simulink library "tailsitter_lib"  (R2018b)
settings: Solver=VariableStepAuto  StartTime=0.0  StopTime=10.0  RelTol=1e-3
undefined symbols (not defined in the file or in its folder): envir, tailsitter
libraries: unit_conversions_lib x2, simple_wing_lib x2, propulsion_lib x2, rotorcraft_lib x2, actuators_lib x2, flightgear_visualization_lib x1, simpleFuselage_lib x1, ground_lib x1, rigidBody_lib x1
settings Model: Creator=Ybeyer  LastModifiedBy=yannic
settings SFSimCC: SimUseLocalCustomCode=off
settings RTWCC: RTWUseLocalCustomCode=off
settings CodeAppCC: StateflowObjectComments=on

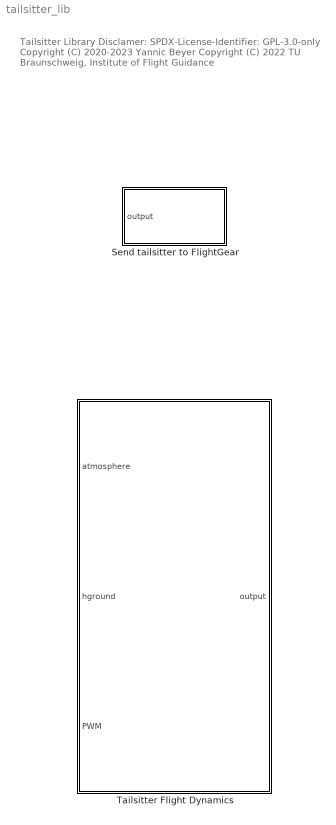
== system tailsitter_lib ==
  note: Tailsitter Library
      |
      | Disclamer:
      | SPDX-License-Identifier: GPL-3.0-only
      |
      | Copyright (C) 2020-2023 Yannic Beyer
      | Copyright (C) 2022 TU Braunschweig, Institute of Flight Guidance
  Send tailsitter to FlightGear : Subsystem  mask{posRef=tailsitter.posRef, IP='127.0.0.1', Port=5502}
      mask prompts: posRef "reference position struct"; IP "FlightGear receive IP"; Port "FlightGear receive Port"
      mask DialogControl DescGroupVar Prompt: Send tailsitter to FlightGear
      mask DialogControl DescTextVar Prompt: Connect the output of the Tailsitter Flight Dynamics block to this block and run a tailsitter FlightGear start script.
  Tailsitter Flight Dynamics : Subsystem  mask{tailsitter=tailsitter}
      mask prompts: tailsitter "tailsitter parameters struct"
      mask DialogControl DescGroupVar Prompt: Tailsitter Flight Dynamics
      mask DialogControl DescTextVar Prompt: For more information about the tailsitter parameters struct see tailsitterLoadParams.

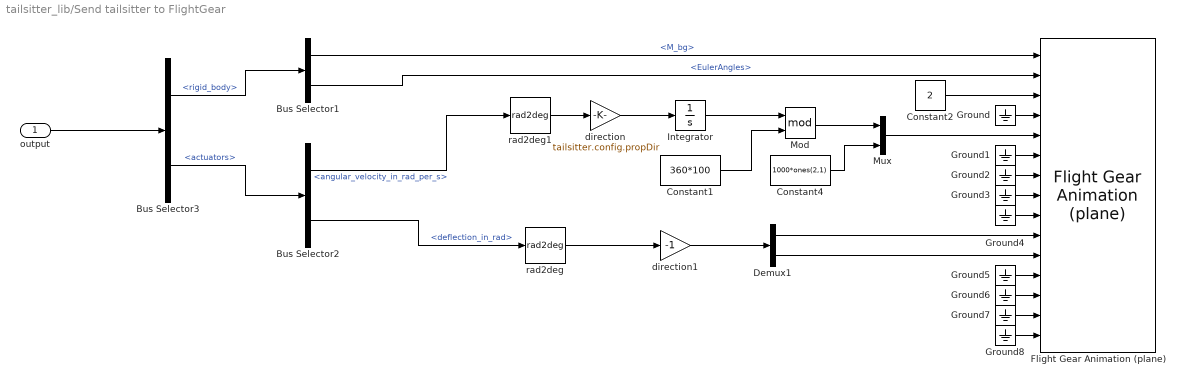
== system tailsitter_lib/Send tailsitter to FlightGear ==
  output : Inport
  Bus Selector1 : BusSelector  OutputSignals=M_bg,EulerAngles
  Bus Selector2 : BusSelector  OutputSignals=angular_velocity_in_rad_per_s,eta_i.deflection_in_rad
  Bus Selector3 : BusSelector  OutputSignals=rigid_body,actuators
  Constant1 : Constant  Value=360*100
  Constant2 : Constant  Value=2
  Constant4 : Constant  Value=1000*ones(2,1)
  Demux1 : Demux  Outputs=2
  Flight Gear Animation (plane) : flightgear_visualization_lib/Flight Gear Animation (plane)  inital_lat=posRef.lat  inital_long=posRef.lon  inital_height=posRef.alt  remoteURL=IP  remotePort=Port
      settings: SourceProductName=LADAC
  Ground{,1..8} (9 alike) : Ground
  Integrator : Integrator
  Mod : Math  Operator=mod  SaturateOnIntegerOverflow=on
  Mux : Mux  Inputs=2
  direction : Gain  Gain=tailsitter.config.propDir
  direction1 : Gain  Gain=-1
  rad2deg : unit_conversions_lib/rad2deg
      settings: SourceProductName=LADAC
  rad2deg1 : unit_conversions_lib/rad2deg
      settings: SourceProductName=LADAC
  wires:
  direction1/1 -> Demux1/1
  Constant4/1 -> Mux/2
  Ground/1 -> Flight Gear Animation (plane)/4
  Demux1/2 -> Flight Gear Animation (plane)/11
  Bus Selector1/2 -> Flight Gear Animation (plane)/2  "<EulerAngles>"
  Demux1/1 -> Flight Gear Animation (plane)/10
  rad2deg1/1 -> direction/1
  Bus Selector1/1 -> Flight Gear Animation (plane)/1  "<M_bg>"
  Ground1/1 -> Flight Gear Animation (plane)/6
  Bus Selector2/2 -> rad2deg/1  "<deflection_in_rad>"
  Bus Selector2/1 -> rad2deg1/1  "<angular_velocity_in_rad_per_s>"
  direction/1 -> Integrator/1
  Mod/1 -> Mux/1
  Integrator/1 -> Mod/1
  Constant1/1 -> Mod/2
  Mux/1 -> Flight Gear Animation (plane)/5
  Constant2/1 -> Flight Gear Animation (plane)/3
  Ground4/1 -> Flight Gear Animation (plane)/9
  rad2deg/1 -> direction1/1
  output/1 -> Bus Selector3/1
  Ground7/1 -> Flight Gear Animation (plane)/14
  Ground6/1 -> Flight Gear Animation (plane)/13
  Ground8/1 -> Flight Gear Animation (plane)/15
  Ground5/1 -> Flight Gear Animation (plane)/12
  Ground2/1 -> Flight Gear Animation (plane)/7
  Ground3/1 -> Flight Gear Animation (plane)/8
  Bus Selector3/1 -> Bus Selector1/1  "<rigid_body>"
  Bus Selector3/2 -> Bus Selector2/1  "<actuators>"

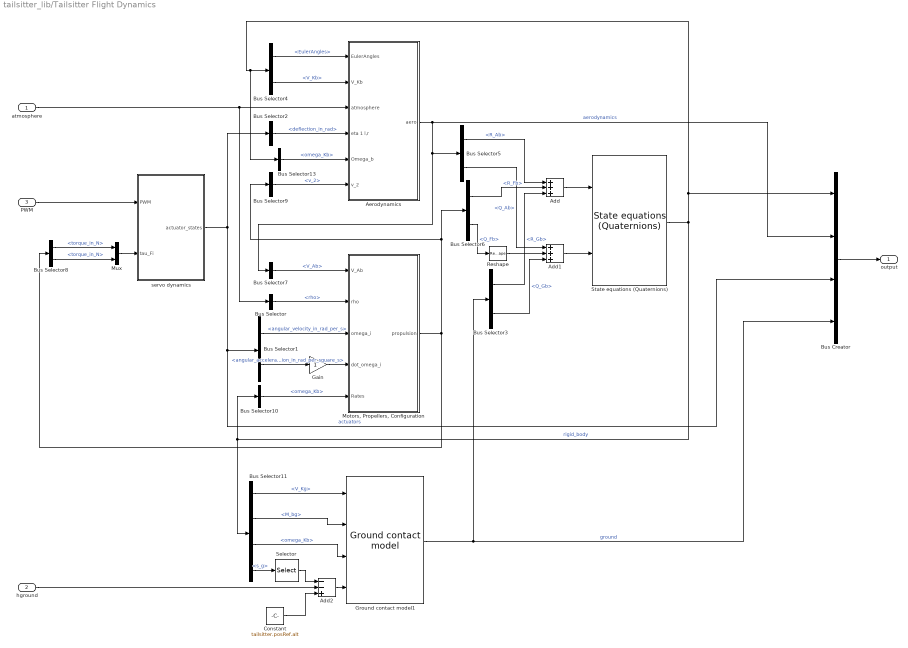
== system tailsitter_lib/Tailsitter Flight Dynamics ==
  atmosphere : Inport
  hground : Inport  Port=2
  PWM : Inport  Port=3
  Add : Sum  Inputs=3
  Add1 : Sum  Inputs=3
  Add2 : Sum  Inputs=--+
  Aerodynamics : Subsystem
  Bus Creator : BusCreator  Inputs=4
  Bus Selector : BusSelector  OutputSignals=athmosphere.rho
  Bus Selector1 : BusSelector  OutputSignals=angular_velocity_in_rad_per_s,angular_acceleration_in_rad_per_square_s
  Bus Selector10 : BusSelector  OutputSignals=omega_Kb
  Bus Selector11 : BusSelector  OutputSignals=V_Kg,M_bg,omega_Kb,s_g
  Bus Selector13 : BusSelector  OutputSignals=omega_Kb
  Bus Selector2 : BusSelector  OutputSignals=eta_i.deflection_in_rad
  Bus Selector3 : BusSelector  OutputSignals=forces_and_moments.R_Gb,forces_and_moments.Q_Gb
  Bus Selector4 : BusSelector  OutputSignals=EulerAngles,V_Kb
  Bus Selector5 : BusSelector  OutputSignals=cg aerodynamics.R_Ab,cg aerodynamics.Q_Ab
  Bus Selector6 : BusSelector  OutputSignals=R_Fb,Q_Fb
  Bus Selector7 : BusSelector  OutputSignals=cg aerodynamics.aeroAxes.V_Ab
  Bus Selector8 : BusSelector  OutputSignals=prop_1.torque_in_N,prop_2.torque_in_N
  Bus Selector9 : BusSelector  OutputSignals=v_2
  Constant : Constant  Value=tailsitter.posRef.alt
  Gain : Gain
  Ground contact model1 : ground_lib/Ground contact model  m=tailsitter.body.m  a_max=tailsitter.grnd.acc_max  xyz_c_hit=tailsitter.config.hitPoints_c  xyz_c_cg=tailsitter.config.CoG_Pos_c  ground_softness_param=tailsitter.grnd.softness_parameter  k_h=tailsitter.grnd.spring_stiffness  k_dot_h=tailsitter.grnd.damping  mu=tailsitter.grnd.friction_coef  k_V=tailsitter.grnd.low_speed_friction_reduction_factor
      settings: SourceProductName=LADAC
  "Motors, Propellers, Configuration" : Subsystem
  Mux : Mux  Inputs=2
  Reshape : Reshape  OutputDimensionality=Column vector (2-D)
  Selector : Selector  InputPortWidth=3  IndexOptions=Index vector (dialog)  Indices=3  OutputSizes=1
  State equations (Quaternions) : rigidBody_lib/State equations (Quaternions)  m=tailsitter.body.m  I=tailsitter.body.I  is_g_checked=off  g=envir.g  omega_Kb_0=tailsitter.ic.omega_kb_b  q_bg_0=tailsitter.ic.q_bg  V_Kb_0=tailsitter.ic.V_kb_b  s_g_0=tailsitter.ic.s_g
      settings: SourceProductName=LADAC
  servo dynamics : Subsystem
  output : Outport
  wires:
  PWM/1 -> servo dynamics/1(PWM)
  atmosphere/1 -> Bus Selector/1, Aerodynamics/3(atmosphere)
  Bus Selector/1 -> "Motors, Propellers, Configuration"/2(rho)  "<rho>"
  servo dynamics/1(actuator_states) -> Bus Creator/3, Bus Selector1/1, Bus Selector2/1  "actuators"
  Bus Selector1/1 -> "Motors, Propellers, Configuration"/3("omega_i ")  "<angular_velocity_in_rad_per_s>"
  Bus Selector1/2 -> Gain/1  "<angular_acceleration_in_rad_per_square_s>"
  Bus Selector2/1 -> Aerodynamics/4(eta 1 l,r)  "<deflection_in_rad>"
  Bus Selector5/1 -> Add/1  "<R_Ab>"
  Bus Selector5/2 -> Add1/1  "<Q_Ab>"
  Bus Selector6/2 -> Reshape/1  "<Q_Fb>"
  Bus Selector6/1 -> Add/2  "<R_Fb>"
  "Motors, Propellers, Configuration"/1(propulsion) -> Bus Selector8/1, Bus Selector9/1, Bus Selector6/1
  Bus Selector7/1 -> "Motors, Propellers, Configuration"/1(V_Ab)  "<V_Ab>"
  Bus Selector8/1 -> Mux/1  "<torque_in_N>"
  Bus Selector9/1 -> Aerodynamics/6(v_2)  "<v_2>"
  Gain/1 -> "Motors, Propellers, Configuration"/4(dot_omega_i)
  Ground contact model1/1 -> Bus Selector3/1, Bus Creator/4  "ground"
  Add1/1 -> State equations (Quaternions)/2
  hground/1 -> Add2/2
  Bus Creator/1 -> output/1
  Add/1 -> State equations (Quaternions)/1
  Aerodynamics/1(aero) -> Bus Selector7/1, Bus Selector5/1, Bus Creator/2  "aerodynamics"
  State equations (Quaternions)/1 -> Bus Selector13/1, Bus Selector4/1, Bus Creator/1, Bus Selector11/1, Bus Selector10/1  "rigid_body"
  Bus Selector4/1 -> Aerodynamics/1("EulerAngles ")  "<EulerAngles>"
  Bus Selector4/2 -> Aerodynamics/2(V_Kb)  "<V_Kb>"
  Bus Selector10/1 -> "Motors, Propellers, Configuration"/5("Rates ")  "<omega_Kb>"
  Bus Selector11/4 -> Selector/1  "<s_g>"
  Bus Selector11/3 -> Ground contact model1/3  "<omega_Kb>"
  Bus Selector11/2 -> Ground contact model1/2  "<M_bg>"
  Bus Selector11/1 -> Ground contact model1/1  "<V_Kg>"
  Bus Selector13/1 -> Aerodynamics/5(Omega_b)  "<omega_Kb>"
  Bus Selector3/2 -> Add1/3  "<Q_Gb>"
  Bus Selector3/1 -> Add/3  "<R_Gb>"
  Reshape/1 -> Add1/2
  Add2/1 -> Ground contact model1/4
  Selector/1 -> Add2/1
  Constant/1 -> Add2/3
  Mux/1 -> servo dynamics/2(tau_Fi)
  Bus Selector8/2 -> Mux/2  "<torque_in_N>"

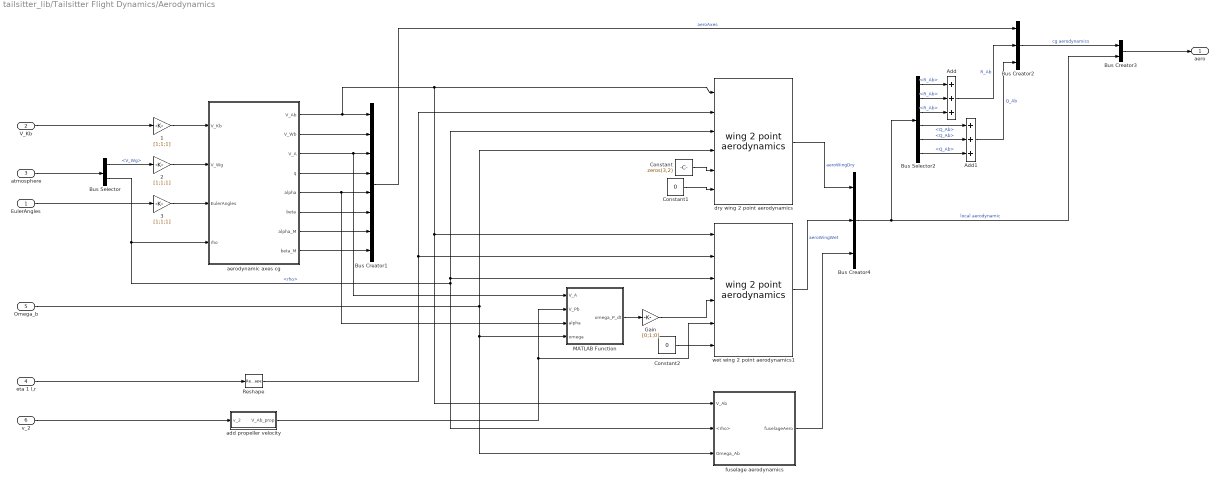
== system tailsitter_lib/Tailsitter Flight Dynamics/Aerodynamics ==
  "EulerAngles " : Inport
  V_Kb : Inport  Port=2
  atmosphere : Inport  Port=3
  eta 1 l,r : Inport  Port=4
  Omega_b : Inport  Port=5
  v_2 : Inport  Port=6
  1 : Gain  Gain=[1;1;1]
  2 : Gain  Gain=[1;1;1]  OutDataTypeStr=double
  3 : Gain  Gain=[1;1;1]
  Add : Sum  Inputs=+++
  Add1 : Sum  Inputs=+++
  Bus Creator1 : BusCreator  Inputs=8
  Bus Creator2 : BusCreator  Inputs=3
  Bus Creator3 : BusCreator  Inputs=2
  Bus Creator4 : BusCreator  Inputs=3
  Bus Selector : BusSelector  OutputSignals=V_Wg,athmosphere.rho
  Bus Selector2 : BusSelector  OutputSignals=aeroWingDry.dynamicsBody.R_Ab,aeroWingWet.dynamicsBody.R_Ab,aeroFuselage.dynamics.R_Ab,aeroWingDry.dynamicsBody.Q_Ab,aeroWingWet.dynamicsBody.Q_Ab,aeroFuselage.dynamics.Q_Ab
  Constant : Constant  Value=zeros(3,2)
  Constant1 : Constant  Value=0
  Constant2 : Constant  Value=0
  Gain : Gain  Gain=[0;1;0]
  MATLAB Function : MATLAB Function  TreatAsAtomicUnit=on
  Reshape : Reshape  OutputDimensionality=Row vector (2-D)
  add propeller velocity : MATLAB Function  TreatAsAtomicUnit=on
  aerodynamic axes cg : MATLAB Function  TreatAsAtomicUnit=on
  dry wing 2 point aerodynamics : simple_wing_lib/wing 2 point aerodynamics  wingStruct=tailsitter.aero.wing  xyz_wing_c=tailsitter.config.xyz_c_wing  xyz_cg_c=tailsitter.config.CoG_Pos_c
      settings: SourceProductName=LADAC
  fuselage aerodynamics : Subsystem  mask{simple_fuselage=tailsitter.aero.fuse}
      mask prompts: simple_fuselage "fuselage struct"
  wet wing 2 point aerodynamics1 : simple_wing_lib/wing 2 point aerodynamics  wingStruct=tailsitter.aero.wing_wet  xyz_wing_c=tailsitter.config.xyz_c_wing  xyz_cg_c=tailsitter.config.CoG_Pos_c
      settings: SourceProductName=LADAC
  aero : Outport
  wires:
  atmosphere/1 -> Bus Selector/1
  Bus Selector/1 -> 2/1  "<V_Wg>"
  2/1 -> aerodynamic axes cg/2(V_Wg)
  "EulerAngles "/1 -> 3/1
  1/1 -> aerodynamic axes cg/1(V_Kb)
  V_Kb/1 -> 1/1
  3/1 -> aerodynamic axes cg/3(EulerAngles)
  aerodynamic axes cg/1(V_Ab) -> Bus Creator1/1, dry wing 2 point aerodynamics/1, fuselage aerodynamics/1(V_Ab), wet wing 2 point aerodynamics1/1
  Bus Selector/2 -> fuselage aerodynamics/2(<rho>), dry wing 2 point aerodynamics/3, wet wing 2 point aerodynamics1/3, aerodynamic axes cg/4(rho)  "<rho>"
  eta 1 l,r/1 -> Reshape/1
  v_2/1 -> add propeller velocity/1(v_2)
  aerodynamic axes cg/2(V_Wb) -> Bus Creator1/2
  aerodynamic axes cg/3(V_A) -> MATLAB Function/1(V_A), Bus Creator1/3
  aerodynamic axes cg/4(q) -> Bus Creator1/4
  aerodynamic axes cg/5(alpha) -> MATLAB Function/3(alpha), Bus Creator1/5
  aerodynamic axes cg/6(beta) -> Bus Creator1/6
  aerodynamic axes cg/7(alpha_M) -> Bus Creator1/7
  aerodynamic axes cg/8(beta_M) -> Bus Creator1/8
  Bus Creator1/1 -> Bus Creator2/1  "aeroAxes"
  Bus Creator2/1 -> Bus Creator3/1  "cg aerodynamics"
  Bus Creator4/1 -> Bus Creator3/2, Bus Selector2/1  "local aerodynamic"
  Bus Creator3/1 -> aero/1
  dry wing 2 point aerodynamics/1 -> Bus Creator4/1  "aeroWingDry"
  wet wing 2 point aerodynamics1/1 -> Bus Creator4/2  "aeroWingWet"
  fuselage aerodynamics/1(fuselageAero) -> Bus Creator4/3
  Bus Selector2/3 -> Add/3  "<R_Ab>"
  Bus Selector2/2 -> Add/2  "<R_Ab>"
  Bus Selector2/1 -> Add/1  "<R_Ab>"
  Bus Selector2/6 -> Add1/3  "<Q_Ab>"
  Bus Selector2/5 -> Add1/2  "<Q_Ab>"
  Bus Selector2/4 -> Add1/1  "<Q_Ab>"
  Add/1 -> Bus Creator2/2  "R_Ab"
  Add1/1 -> Bus Creator2/3  "Q_Ab"
  Reshape/1 -> dry wing 2 point aerodynamics/2, wet wing 2 point aerodynamics1/2
  Constant/1 -> dry wing 2 point aerodynamics/5
  add propeller velocity/1(V_Ab_prop) -> MATLAB Function/2(V_Pb), wet wing 2 point aerodynamics1/5
  Omega_b/1 -> MATLAB Function/4(omega), fuselage aerodynamics/3(Omega_Ab), dry wing 2 point aerodynamics/4
  MATLAB Function/1(omega_P_dt) -> Gain/1
  Gain/1 -> wet wing 2 point aerodynamics1/4
  Constant1/1 -> dry wing 2 point aerodynamics/6
  Constant2/1 -> wet wing 2 point aerodynamics1/6

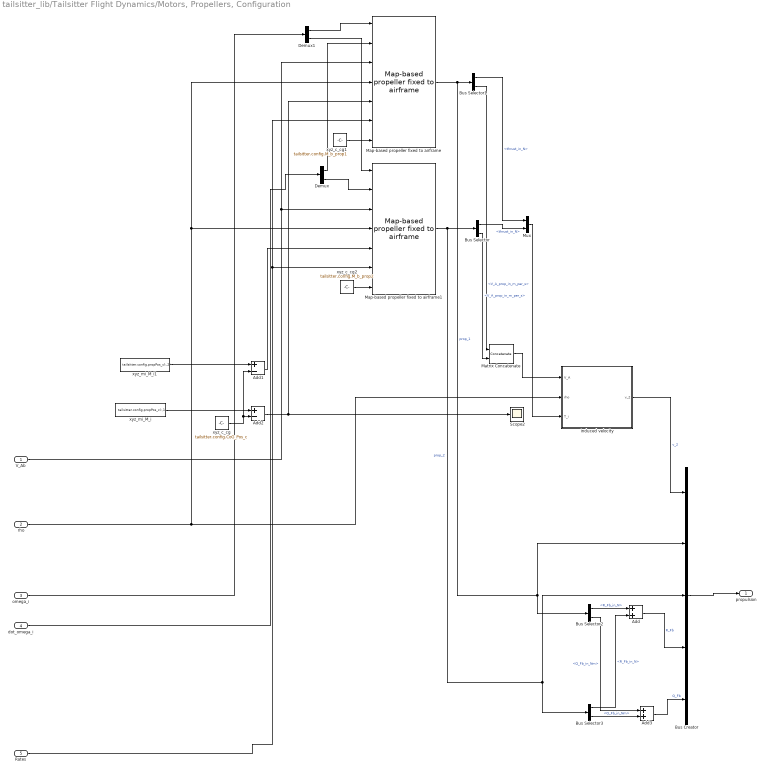
== system tailsitter_lib/Tailsitter Flight Dynamics/Motors, Propellers, Configuration ==
  V_Ab : Inport
  rho : Inport  Port=2
  "omega_i " : Inport  Port=3
  dot_omega_i : Inport  Port=4
  "Rates " : Inport  Port=5
  Add : Sum
  Add1 : Sum  Inputs=+-
  Add2 : Sum  Inputs=+-
  Add3 : Sum
  Bus Creator : BusCreator  Inputs=5
  Bus Selector : BusSelector  OutputSignals=thrust_in_N,V_A_prop_in_m_per_s
  Bus Selector1 : BusSelector  OutputSignals=thrust_in_N,V_A_prop_in_m_per_s
  Bus Selector2 : BusSelector  OutputSignals=R_Fb_in_N,Q_Fb_in_Nm
  Bus Selector3 : BusSelector  OutputSignals=R_Fb_in_N,Q_Fb_in_Nm
  Demux : Demux  Outputs=2
  Demux1 : Demux  Outputs=2
  Map-based propeller fixed to airframe : propulsion_lib/Map-based propeller fixed to airframe  prop_map_fit=tailsitter.prop.map_fit  I_prop=tailsitter.prop.I  rotation_orientation=tailsitter.config.propDir(1)
      settings: SourceProductName=LADAC
  Map-based propeller fixed to airframe1 : propulsion_lib/Map-based propeller fixed to airframe  prop_map_fit=tailsitter.prop.map_fit  I_prop=tailsitter.prop.I  rotation_orientation=tailsitter.config.propDir(2)
      settings: SourceProductName=LADAC
  Matrix Concatenate : Concatenate  Mode=Multidimensional array  ConcatenateDimension=2
  Mux : Mux  Inputs=2
  Scope2 : Scope
  induced velocity : Subsystem
  xyz_c_cg : Constant  Value=tailsitter.config.CoG_Pos_c
  xyz_c_cg1 : Constant  Value=tailsitter.config.M_b_prop1
  xyz_c_cg2 : Constant  Value=tailsitter.config.M_b_prop2
  xyz_mi_M_i : Constant  Value=tailsitter.config.propPos_c(:,1)
  xyz_mi_M_i1 : Constant  Value=tailsitter.config.propPos_c(:,2)
  propulsion : Outport
  wires:
  V_Ab/1 -> Map-based propeller fixed to airframe1/3, Map-based propeller fixed to airframe/3
  "Rates "/1 -> Map-based propeller fixed to airframe/6, Map-based propeller fixed to airframe1/6
  rho/1 -> Map-based propeller fixed to airframe1/4, Map-based propeller fixed to airframe/4, induced velocity/2(rho)
  dot_omega_i/1 -> Demux/1
  "omega_i "/1 -> Demux1/1
  xyz_mi_M_i/1 -> Add2/1
  Add2/1 -> Map-based propeller fixed to airframe/5, Scope2/1
  xyz_c_cg/1 -> Add1/2, Add2/2
  Bus Creator/1 -> propulsion/1
  induced velocity/1(v_2) -> Bus Creator/1  "v_2"
  xyz_c_cg1/1 -> Map-based propeller fixed to airframe/7
  xyz_c_cg2/1 -> Map-based propeller fixed to airframe1/7
  xyz_mi_M_i1/1 -> Add1/1
  Add1/1 -> Map-based propeller fixed to airframe1/5
  Demux/2 -> Map-based propeller fixed to airframe1/2
  Demux/1 -> Map-based propeller fixed to airframe/2
  Demux1/1 -> Map-based propeller fixed to airframe/1
  Demux1/2 -> Map-based propeller fixed to airframe1/1
  Map-based propeller fixed to airframe1/1 -> Bus Selector3/1, Bus Creator/3, Bus Selector/1  "prop_2"
  Mux/1 -> induced velocity/3(T_i)
  Bus Selector/1 -> Mux/2  "<thrust_in_N>"
  Map-based propeller fixed to airframe/1 -> Bus Selector2/1, Bus Creator/2, Bus Selector1/1  "prop_1"
  Bus Selector1/1 -> Mux/1  "<thrust_in_N>"
  Bus Selector/2 -> Matrix Concatenate/2  "<V_A_prop_in_m_per_s>"
  Bus Selector1/2 -> Matrix Concatenate/1  "<V_A_prop_in_m_per_s>"
  Matrix Concatenate/1 -> induced velocity/1(V_A)
  Bus Selector3/2 -> Add3/2  "<Q_Fb_in_Nm>"
  Bus Selector2/2 -> Add3/1  "<Q_Fb_in_Nm>"
  Add3/1 -> Bus Creator/5  "Q_Fb"
  Bus Selector2/1 -> Add/1  "<R_Fb_in_N>"
  Bus Selector3/1 -> Add/2  "<R_Fb_in_N>"
  Add/1 -> Bus Creator/4  "R_Fb"

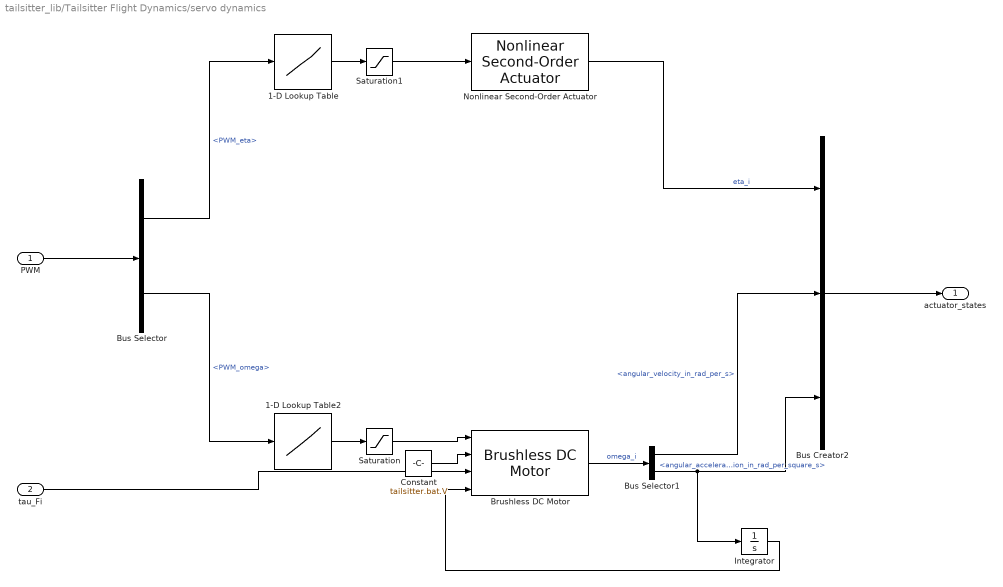
== system tailsitter_lib/Tailsitter Flight Dynamics/servo dynamics ==
  PWM : Inport
  tau_Fi : Inport  Port=2
  1-D Lookup Table : Lookup_n-D  NumberOfTableDimensions=1  BreakpointsForDimension1=[1100;1900]  Table=[tailsitter.act.elevons.deflectionMin;tailsitter.act.elevons.deflectionMax]  InternalRulePriority=Speed  RndMeth=Simplest  InputSameDT=on
  1-D Lookup Table2 : Lookup_n-D  NumberOfTableDimensions=1  BreakpointsForDimension1=[1000;2000]  Table=[0;1]  InternalRulePriority=Speed  RndMeth=Simplest  InputSameDT=on
  Brushless DC Motor : actuators_lib/Brushless DC Motor  K_T=tailsitter.motor.KT  J_prop=tailsitter.prop.I  R_i=tailsitter.motor.R  IC_omega=0  omega_max=Inf  omega_min=0
      settings: SourceProductName=LADAC
  Bus Creator2 : BusCreator  Inputs=3
  Bus Selector : BusSelector  OutputSignals=PWM_eta,PWM_omega
  Bus Selector1 : BusSelector  OutputSignals=angular_velocity_in_rad_per_s,angular_acceleration_in_rad_per_square_s
  Constant : Constant  Value=tailsitter.bat.V
  Integrator : Integrator  InitialCondition=tailsitter.ic.motor_speed
  Nonlinear Second-Order Actuator : actuators_lib/Nonlinear Second-Order Actuator  omega=tailsitter.act.elevons.naturalFrequency  d=tailsitter.act.elevons.dampingRatio  A_max=tailsitter.act.elevons.deflectionMax  A_min=tailsitter.act.elevons.deflectionMin  dot_A_max=tailsitter.act.elevons.deflectionRateMax  dot_A_min=-tailsitter.act.elevons.deflectionRateMax  A_0=tailsitter.ic.eta  dot_A_0=tailsitter.ic.dot_eta
      settings: SourceProductName=LADAC
  Saturation : Saturate  UpperLimit=1  LowerLimit=0
  Saturation1 : Saturate  UpperLimit=tailsitter.act.elevons.deflectionMax  LowerLimit=tailsitter.act.elevons.deflectionMin
  actuator_states : Outport
  wires:
  Brushless DC Motor/1 -> Bus Selector1/1  "omega_i"
  tau_Fi/1 -> Brushless DC Motor/3
  Saturation/1 -> Brushless DC Motor/1
  1-D Lookup Table/1 -> Saturation1/1
  Saturation1/1 -> Nonlinear Second-Order Actuator/1
  1-D Lookup Table2/1 -> Saturation/1
  PWM/1 -> Bus Selector/1
  Bus Selector/1 -> 1-D Lookup Table/1  "<PWM_eta>"
  Bus Creator2/1 -> actuator_states/1
  Nonlinear Second-Order Actuator/1 -> Bus Creator2/1  "eta_i"
  Bus Selector/2 -> 1-D Lookup Table2/1  "<PWM_omega>"
  Constant/1 -> Brushless DC Motor/2
  Bus Selector1/2 -> Bus Creator2/3, Integrator/1  "<angular_acceleration_in_rad_per_square_s>"
  Integrator/1 -> Brushless DC Motor/4
  Bus Selector1/1 -> Bus Creator2/2  "<angular_velocity_in_rad_per_s>"

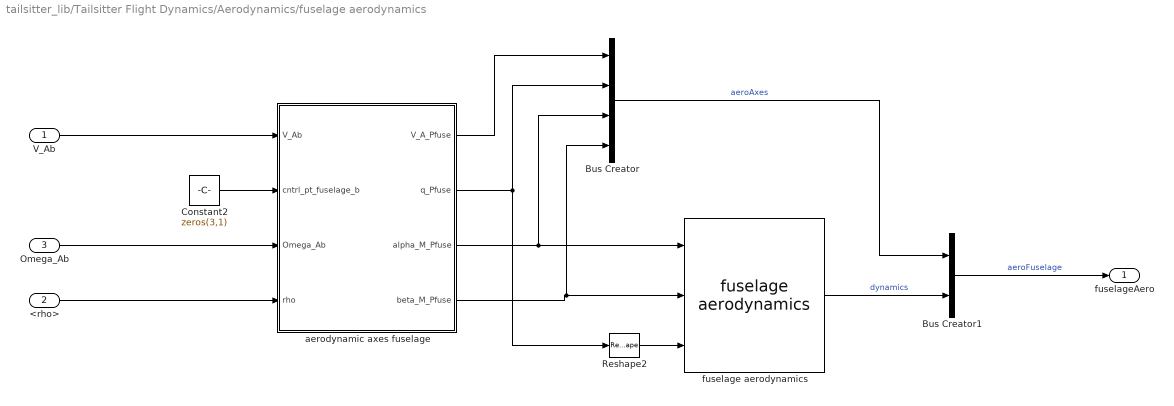
== system tailsitter_lib/Tailsitter Flight Dynamics/Aerodynamics/fuselage aerodynamics ==
  V_Ab : Inport
  <rho> : Inport  Port=2
  Omega_Ab : Inport  Port=3
  Bus Creator : BusCreator  Inputs=4
  Bus Creator1 : BusCreator  Inputs=2
  Constant2 : Constant  Value=zeros(3,1)
  Reshape2 : Reshape  OutputDimensionality=Row vector (2-D)
  aerodynamic axes fuselage : MATLAB Function  TreatAsAtomicUnit=on
  fuselage aerodynamics : simpleFuselage_lib/fuselage aerodynamics  simple_fuselage=simple_fuselage
      settings: SourceProductName=LADAC
  fuselageAero : Outport
  wires:
  aerodynamic axes fuselage/3(alpha_M_Pfuse) -> Bus Creator/3, fuselage aerodynamics/1
  Constant2/1 -> aerodynamic axes fuselage/2(cntrl_pt_fuselage_b)
  Reshape2/1 -> fuselage aerodynamics/3
  aerodynamic axes fuselage/4(beta_M_Pfuse) -> Bus Creator/4, fuselage aerodynamics/2
  Omega_Ab/1 -> aerodynamic axes fuselage/3(Omega_Ab)
  V_Ab/1 -> aerodynamic axes fuselage/1(V_Ab)
  aerodynamic axes fuselage/1(V_A_Pfuse) -> Bus Creator/1
  <rho>/1 -> aerodynamic axes fuselage/4(rho)
  aerodynamic axes fuselage/2(q_Pfuse) -> Reshape2/1, Bus Creator/2
  Bus Creator/1 -> Bus Creator1/1  "aeroAxes"
  fuselage aerodynamics/1 -> Bus Creator1/2  "dynamics"
  Bus Creator1/1 -> fuselageAero/1  "aeroFuselage"

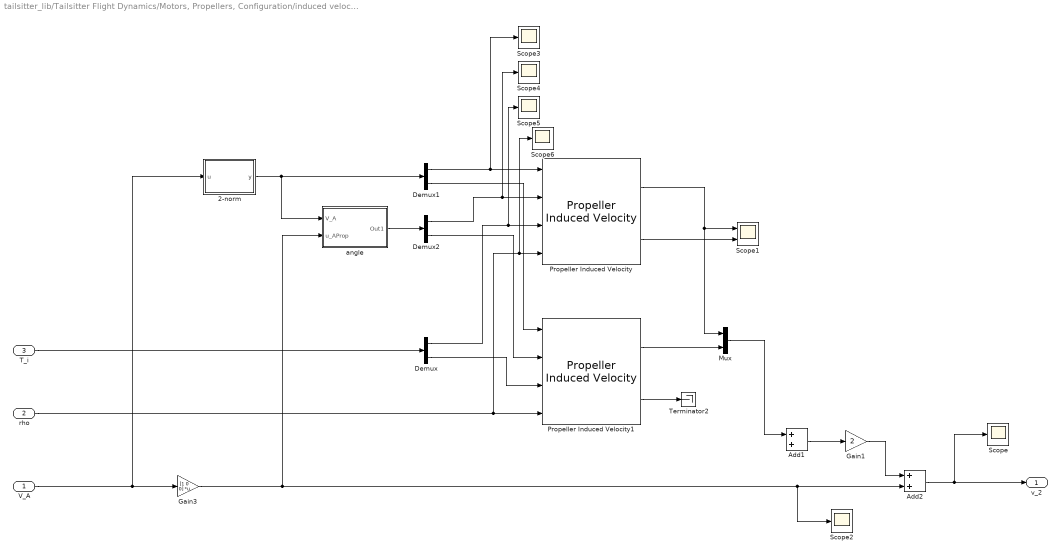
== system tailsitter_lib/Tailsitter Flight Dynamics/Motors, Propellers, Configuration/induced velocity ==
  V_A : Inport
  rho : Inport  Port=2
  T_i : Inport  Port=3
  2-norm : MATLAB Function  TreatAsAtomicUnit=on
  Add1 : Sum
  Add2 : Sum
  Demux : Demux  Outputs=2
  Demux1 : Demux  Outputs=2
  Demux2 : Demux  Outputs=2
  Gain1 : Gain  Gain=2
  Gain3 : Gain  Gain=[1 0 0]  Multiplication=Matrix(K*u)
  Mux : Mux  Inputs=2
  Propeller Induced Velocity : rotorcraft_lib/Propeller Induced Velocity  F=(str2num(tailsitter.prop.name(1))*0.0254/2)^2*pi
      settings: SourceProductName=LADAC
  Propeller Induced Velocity1 : rotorcraft_lib/Propeller Induced Velocity  F=(str2num(tailsitter.prop.name(1))*0.0254/2)^2*pi
      settings: SourceProductName=LADAC
  Scope{,2..6} (6 alike) : Scope
  Scope1 : Scope  NumInputPorts=2
  Terminator2 : Terminator
  angle : Subsystem
  v_2 : Outport
  wires:
  T_i/1 -> Demux/1
  rho/1 -> Scope6/1, Propeller Induced Velocity/4, Propeller Induced Velocity1/4
  2-norm/1(y) -> angle/1(V_A), Demux1/1
  V_A/1 -> 2-norm/1(u), Gain3/1
  Demux/1 -> Scope5/1, Propeller Induced Velocity/3
  Demux2/1 -> Scope4/1, Propeller Induced Velocity/2
  Demux1/2 -> Propeller Induced Velocity1/1
  Demux2/2 -> Propeller Induced Velocity1/2
  Demux/2 -> Propeller Induced Velocity1/3
  Propeller Induced Velocity/1 -> Mux/1, Scope1/1
  Propeller Induced Velocity1/1 -> Mux/2
  Add2/1 -> Scope/1, v_2/1
  Add1/1 -> Gain1/1
  Gain3/1 -> Add2/2, Scope2/1, angle/2(u_AProp)
  Gain1/1 -> Add2/1
  Mux/1 -> Add1/1
  Propeller Induced Velocity/2 -> Scope1/2
  Propeller Induced Velocity1/2 -> Terminator2/1
  angle/1(Out1) -> Demux2/1
  Demux1/1 -> Scope3/1, Propeller Induced Velocity/1

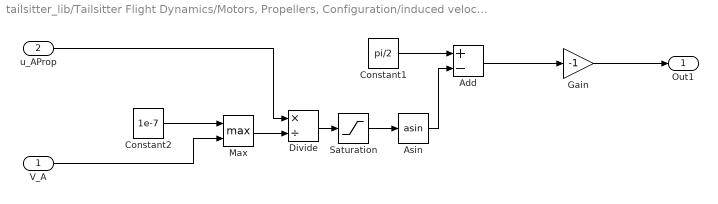
== system tailsitter_lib/Tailsitter Flight Dynamics/Motors, Propellers, Configuration/induced velocity/angle ==
  V_A : Inport
  u_AProp : Inport  Port=2
  Add : Sum  Inputs=+-
  Asin : Trigonometry  Operator=asin  OutputSignalType=real
  Constant1 : Constant  Value=pi/2
  Constant2 : Constant  Value=1e-7
  Divide : Product  Inputs=*/
  Gain : Gain  Gain=-1
  Max : MinMax  Function=max  Inputs=2
  Saturation : Saturate  UpperLimit=0.99  LowerLimit=-0.99
  Out1 : Outport
  wires:
  V_A/1 -> Max/2
  Max/1 -> Divide/2
  u_AProp/1 -> Divide/1
  Add/1 -> Gain/1
  Divide/1 -> Saturation/1
  Asin/1 -> Add/2
  Constant1/1 -> Add/1
  Constant2/1 -> Max/1
  Gain/1 -> Out1/1
  Saturation/1 -> Asin/1

== matlab function tailsitter_lib/Tailsitter Flight Dynamics/Motors, Propellers, Configuration/induced velocity/2-norm ==
  data: u input; y output
function y = fcn(u)
y=vecnorm(u,2,1);

== matlab function tailsitter_lib/Tailsitter Flight Dynamics/Aerodynamics/aerodynamic axes cg ==
  data: V_Kb input; V_Ab output; V_Wb output; V_A output; q output; alpha output; beta output; V_Wg input; EulerAngles input; alpha_M output; beta_M output; rho input
function [ V_Ab, V_Wb, V_A, q, alpha, beta, alpha_M, beta_M ] = ...
    fcn( V_Kb, V_Wg, EulerAngles, rho ) %#codegen

% compute rotation matrix from g to b frame
M_bg = euler2Dcm( EulerAngles );

% compute velocities
V_Wb = M_bg * V_Wg;
V_Ab = V_Kb - V_Wb;

% calculate aerodynamic speed (TAS) and dynamic pressure
V_A = norm( V_Ab, 2 );
q   = rho/2 * V_A^2;

% compute aerodynamic angles
[ alpha, beta ] = aeroAngles( V_Ab );

% compute modified aerodynamic angles
[ alpha_M, beta_M ] = aeroAnglesMod( V_Ab );
 
end

== matlab function tailsitter_lib/Tailsitter Flight Dynamics/Aerodynamics/fuselage aerodynamics/aerodynamic axes fuselage ==
  data: V_Ab input; cntrl_pt_fuselage_b input; Omega_Ab input; V_A_Pfuse output; q_Pfuse output; alpha_M_Pfuse output; beta_M_Pfuse output; rho input
function [ V_A_Pfuse, q_Pfuse, alpha_M_Pfuse, beta_M_Pfuse ] = fcn( V_Ab, ...
    cntrl_pt_fuselage_b, Omega_Ab, rho )
%#codegen

% compute inflow at specified points
V_Ab_Pfuse = velocityFromRot( V_Ab, Omega_Ab, cntrl_pt_fuselage_b );
V_A_Pfuse = real( max( 0, sqrt(V_Ab_Pfuse(1,:).^2 + V_Ab_Pfuse(2,:).^2 + V_Ab_Pfuse(3,:).^2) ) );
q_Pfuse = rho/2 * V_A_Pfuse.^2;
[ alpha_M_Pfuse, beta_M_Pfuse ] = aeroAnglesMod( V_Ab_Pfuse );

end

== matlab function tailsitter_lib/Tailsitter Flight Dynamics/Aerodynamics/add propeller velocity ==
  data: V_Ab_prop output; v_2 input
function V_Ab_prop = fcn( v_2 ) %#codegen
    V_Ab_prop = [ v_2; zeros( 2, length(v_2) ) ];
end

== matlab function tailsitter_lib/Tailsitter Flight Dynamics/Aerodynamics/MATLAB Function ==
  data: V_A input; V_Pb input; alpha input; omega input; omega_P_dt output
function omega_P_dt = fcn(V_A, V_Pb, alpha, omega)

V_P = mean(sqrt(V_Pb(1,:).^2+V_Pb(3,:).^2));

k = V_A / max(1e-5, sqrt(V_P^2+V_A^2));

omega_P_dt = k*cos(alpha)/(sqrt(1-k^2*(sin(alpha))^2))*omega(2);

end
